simulink model "simulator_model_controller_impedance3"  (R2023b)
settings: Solver=ode4  StartTime=0.0  StopTime=10  FixedStep=0.01  RelTol=1e-3
values from neighbouring files (symbols this model uses):
  Fc = Simulink.Parameter([0; 0])    [main.m]
  Fv = 0.04    [main.m]
  g = Simulink.Parameter(9.81)    [main.m]
  I1 = Simulink.Parameter( (1/12)*m1.Value*(l1.Value^2) )    [main.m]
  I2 = Simulink.Parameter( (1/12)*m2.Value*(l2.Value^2) )    [main.m]
  K = 1000    [main.m]    (also in symbolic_functions.m = simplify(1/2*dq'*M*dq))
  ke = Simulink.Parameter([Ks 0 ; 0 Ks])    [main.m]
  kp = Simulink.Parameter([0 0 ; 0 10000])    [main.m]
  l1 = Simulink.Parameter(1)    [main.m]    (also in plot_robot.m = inputs(3); plot_robot_3links.m = inputs(4))
  l2 = Simulink.Parameter(1)    [main.m]    (also in plot_robot.m = inputs(4); plot_robot_3links.m = inputs(5))
  lc1 = Simulink.Parameter(l1.Value/2)    [main.m]
  lc2 = Simulink.Parameter(l2.Value/2)    [main.m]
  m1 = Simulink.Parameter(0.5)    [main.m]
  m2 = Simulink.Parameter(0.2)    [main.m]
  Xe = Simulink.Parameter([0.2 ; -0.2])    [main.m]
settings Model: Creator=Gabriel  LastModifiedBy=Bruno

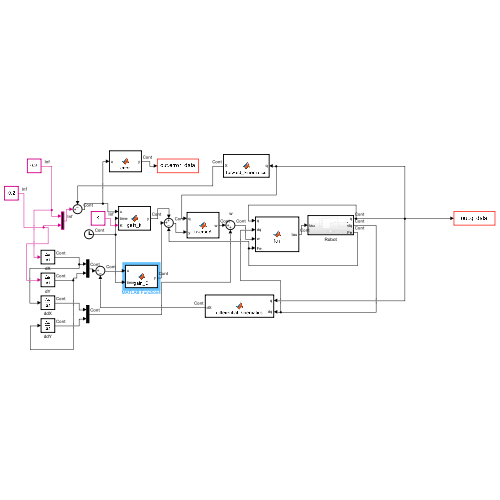
[thumbnail: Simulink's stored preview of the top-level diagram]
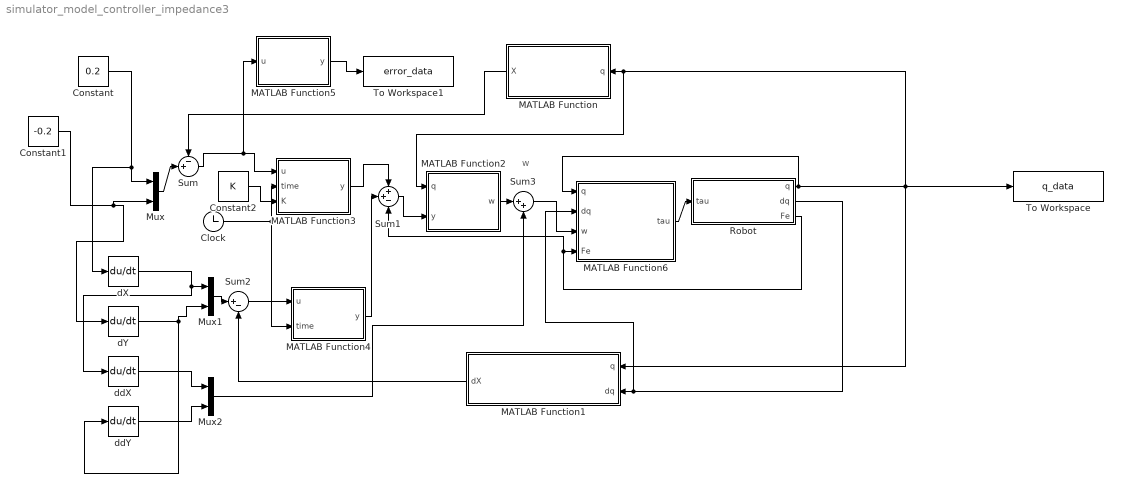
== system simulator_model_controller_impedance3 ==
  note: w
  Clock : Clock
  Constant : Constant  Value=0.2
  Constant1 : Constant  Value=-0.2
  Constant2 : Constant  Value=K
  MATLAB Function : MATLAB Function  TreatAsAtomicUnit=on
  MATLAB Function1 : MATLAB Function  TreatAsAtomicUnit=on
  MATLAB Function2 : MATLAB Function  TreatAsAtomicUnit=on
  MATLAB Function3 : MATLAB Function  TreatAsAtomicUnit=on
  MATLAB Function4 : MATLAB Function  TreatAsAtomicUnit=on
  MATLAB Function5 : MATLAB Function  TreatAsAtomicUnit=on
  MATLAB Function6 : MATLAB Function  TreatAsAtomicUnit=on
  Mux : Mux  Inputs=2
  Mux1 : Mux  Inputs=2
  Mux2 : Mux  Inputs=2
  Robot : Subsystem
  Sum : Sum  Inputs=-+|
  Sum1 : Sum  Inputs=++-
  Sum2 : Sum  Inputs=|+-
  Sum3 : Sum  Inputs=|++
  To Workspace : ToWorkspace  VariableName=q_data  SampleTime=-1
      settings: Save2DSignal=2-D array (concatenate along first dimension)
  To Workspace1 : ToWorkspace  VariableName=error_data  SampleTime=-1
      settings: Save2DSignal=2-D array (concatenate along first dimension)
  dX : Derivative
  dY : Derivative
  ddX : Derivative
  ddY : Derivative
  wires:
  Constant1/1 -> dY/1, Mux/2
  Robot/1(q) -> MATLAB Function6/1(q), MATLAB Function2/1(q), MATLAB Function/1(q), To Workspace/1, MATLAB Function1/1(q)
  MATLAB Function6/1(tau) -> Robot/1(tau)
  Robot/3(Fe) -> Sum1/3, MATLAB Function6/4(Fe)
  Robot/2(dq) -> MATLAB Function6/2(dq), MATLAB Function1/2(dq)
  Sum1/1 -> MATLAB Function2/2(y)
  MATLAB Function2/1(w) -> Sum3/1
  Sum3/1 -> MATLAB Function6/3(w)
  dX/1 -> ddX/1, Mux1/1
  dY/1 -> Mux1/2, ddY/1
  ddX/1 -> Mux2/1
  ddY/1 -> Mux2/2
  Mux2/1 -> Sum3/2
  Clock/1 -> MATLAB Function4/2(time), MATLAB Function3/2(time)
  MATLAB Function3/1(y) -> Sum1/1
  Mux/1 -> Sum/2
  MATLAB Function/1(X) -> Sum/1
  Mux1/1 -> Sum2/1
  MATLAB Function1/1(dX) -> Sum2/2
  MATLAB Function4/1(y) -> Sum1/2
  Constant/1 -> dX/1, Mux/1
  Sum2/1 -> MATLAB Function4/1(u)
  Sum/1 -> MATLAB Function5/1(u), MATLAB Function3/1(u)
  Constant2/1 -> MATLAB Function3/3(K)
  MATLAB Function5/1(y) -> To Workspace1/1

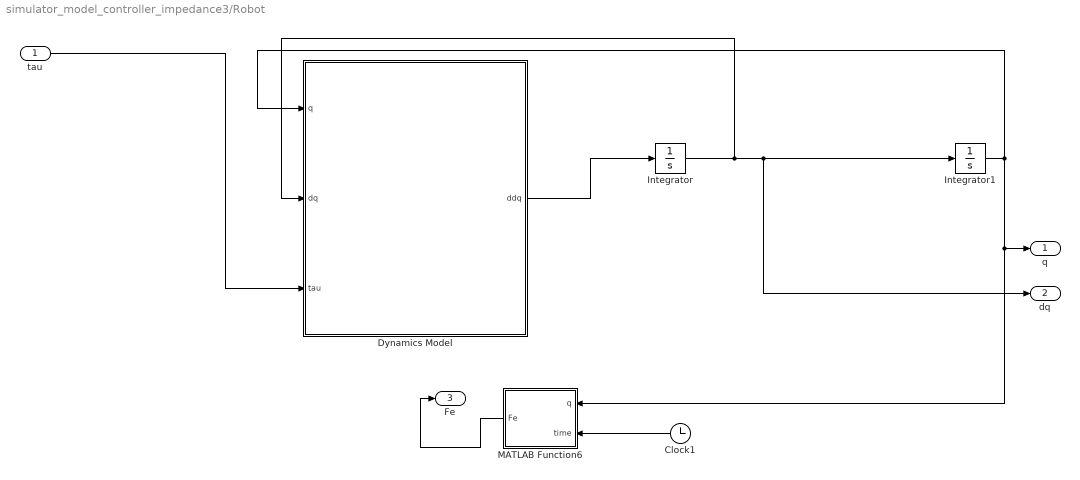
== system simulator_model_controller_impedance3/Robot ==
  tau : Inport
  Clock1 : Clock
  Dynamics Model : MATLAB Function  TreatAsAtomicUnit=on
  Integrator : Integrator  InitialCondition=[0;0]
  Integrator1 : Integrator  InitialCondition=[pi/2;pi/4]
  MATLAB Function6 : MATLAB Function  TreatAsAtomicUnit=on
  q : Outport
  dq : Outport  Port=2
  Fe : Outport  Port=3
  wires:
  Integrator1/1 -> MATLAB Function6/1(q), q/1, Dynamics Model/1(q)
  tau/1 -> Dynamics Model/3(tau)
  Dynamics Model/1(ddq) -> Integrator/1
  Integrator/1 -> Dynamics Model/2(dq), dq/1, Integrator1/1
  MATLAB Function6/1(Fe) -> Fe/1
  Clock1/1 -> MATLAB Function6/2(time)

== matlab function simulator_model_controller_impedance3/MATLAB Function5 ==
  data: u input; y output
function y = error(u)
theta = atan(-1);
R = [cos(theta) -sin(theta); sin(theta) cos(theta)];


y = R' * u;

== matlab function simulator_model_controller_impedance3/MATLAB Function6 ==
  data: q input; tau output; dq input; w input; m1 parameter; m2 parameter; l1 parameter; l2 parameter; lc1 parameter; lc2 parameter; I1 parameter; I2 parameter; g parameter; Fe input
function tau = fcn(q,dq,w, m1, m2, l1, l2, lc1, lc2, I1, I2, g,Fe)
G = gravity_vector(q(1),q(2),m1,m2,l1,l2,lc1,lc2,g);
J = Jacobian.linear_jacobian(q(1),q(2),l1,l2);
M = mass_matrix(q(1),q(2),m1,m2,l1,l2,lc1,lc2,I1,I2);
C = coriolis_matrix(q(1),q(2),dq(1),dq(2),m1,m2,l1,l2,lc1,lc2);
dJ = Jacobian.differential_jacobian(q(1),q(2),dq(1),dq(2),l1,l2);

%torquec= zeta + G + C*dq+J'*Fe;
torquec= M * (J \ (w - dJ*dq)) + (G + C*dq)+J'*Fe;
tau = torquec - J'*Fe; 



%F = (eye(2)-Ma/Md)*Fe + (Da-Dd*Ma/Md)*dX + (Ka - Ma/Md*Kd)*X + Ma/Md*(Dd*dXd + Kd*Xd);

== matlab function simulator_model_controller_impedance3/Robot/MATLAB Function6 ==
  data: q input; Fe output; time input; l1 parameter; l2 parameter; Xe parameter; Fc parameter; kp parameter; ke parameter
function Fe = force(q, time, l1, l2, Xe, Fc, kp, ke)
    % Posição do end-effector
    X = forward_kinematics(q(1), q(2), l1, l2);

    %if (X(2) <= Xe(2) && X(1) >= Xe(1))   % end-effector abaixo da superfície do osso
    if (X(1) >= Xe(1) && X(2) <= Xe(2))
        % Calcular força de contacto
        Fe_compliance = [ke(1,1)*(X(1)-Xe(1)); ke(2,2)*(X(2)-Xe(2))];
    else
        % Sem contacto
        Fe_compliance = [0; 0];
    end
    if time >= 1
        F_surgeon = [370;-370];    
    else 
        F_surgeon = [0;0];
    end

    % Soma de todas as forças
    Fe = Fe_compliance - F_surgeon;
end

== matlab function simulator_model_controller_impedance3/Robot/Dynamics Model ==
  data: q input; ddq output; dq input; tau input; m1 parameter; m2 parameter; l1 parameter; l2 parameter; lc1 parameter; lc2 parameter; I1 parameter; I2 parameter; g parameter; Fv parameter
function ddq = dynamics(q,dq,tau,m1, m2, l1, l2, lc1, lc2, I1, I2, g, Fv)

    M = mass_matrix(q(1),q(2),m1,m2,l1,l2,lc1,lc2,I1,I2);
    C = coriolis_matrix(q(1),q(2),dq(1),dq(2),m1,m2,l1,l2,lc1,lc2);
    G = gravity_vector(q(1),q(2),m1,m2,l1,l2,lc1,lc2,g);
    
    %--------------------------------------------
    %     REGULARIZAÇÃO PARA EVITAR SINGULARIDADES
    %--------------------------------------------
    cond_min = 1e-6;       % limite antes de considerar a matriz perigosa
    eps_reg  = 1e-6;       % força de regularização

    if rcond(M) < cond_min
        M = M + eps_reg * eye(2);
    end

    %--------------------------------------------
    %     CÁLCULO DAS ACELERAÇÕES
    %--------------------------------------------
    ddq = M \ (tau - C*dq - G - Fv*dq);

    %--------------------------------------------
    %     LIMITAÇÃO PARA EVITAR EXPLOSÕES NUMÉRICAS
    %--------------------------------------------
    ddq_max = 1e4;
    ddq = min(max(ddq, -ddq_max), ddq_max);

end

== matlab function simulator_model_controller_impedance3/MATLAB Function ==
  data: q input; l1 parameter; X output; l2 parameter
function X  = forward_kinematics(q, l1,l2)
    X=forward_kinematics(q(1),q(2),l1,l2);

== matlab function simulator_model_controller_impedance3/MATLAB Function1 ==
  data: q input; dX output; dq input; l1 parameter; l2 parameter
function dX  = differential_kinematics(q,dq, l1, l2)
            q1=q(1);
            q2=q(2);
            J=Jacobian.linear_jacobian(q1,q2,l1,l2);
            dX = J*dq;

== matlab function simulator_model_controller_impedance3/MATLAB Function2 ==
  data: w output; q input; m1 parameter; m2 parameter; l1 parameter; l2 parameter; lc1 parameter; lc2 parameter; I1 parameter; I2 parameter; y input
function w = inverseA(q, m1, m2, l1, l2, lc1, lc2, I1, I2,y)
J = Jacobian.linear_jacobian(q(1),q(2),l1,l2);
M = mass_matrix(q(1),q(2),m1,m2,l1,l2,lc1,lc2,I1,I2);
invA = (J*inv(M)*J')/10;
w = invA*y;

== matlab function simulator_model_controller_impedance3/MATLAB Function3 ==
  data: u input; y output; time input; kp parameter; K input
function y = gain_k(u,time, kp, K)
theta = atan(-1); 
R = [cos(theta) -sin(theta); sin(theta) cos(theta)];
K_task = R * kp * R';
if time <1
    y=K*u;
else
    y=K_task*u;
end

== matlab function simulator_model_controller_impedance3/MATLAB Function4 ==
  data: u input; y output; time input; Dd parameter
function y = gain_D(u,time, Dd)
theta = atan(-1);
R = [cos(theta) -sin(theta); sin(theta) cos(theta)];

D_task = diag([sqrt(7000/3)*3, sqrt(7000/3)*3]);
D = R * D_task * R';

if time <1
    y=[sqrt(1000/3)*9 0; 0 sqrt(1000/3)*9]*u;
else
    y=D*u;
end
